simulink model "HPP"  (R2026a)
settings: Solver=ode1  StopTime=p.sim.Tstop  FixedStep=HPP_Tnet
model workspace (MAT data in the model file):
  HPP_Tnet = 0.001
  HPP_Ts = 0.001
  HPP_delays = 1
  HPP_f0 = 50
  HPP_network = 1
  HPP_simscape = 1
  buildInfo : object (value not decoded)
undefined symbols (not defined in the file): p
libraries: ee_lib x57, nesl_utility x29, fl_lib x6
(part 4 of 5)

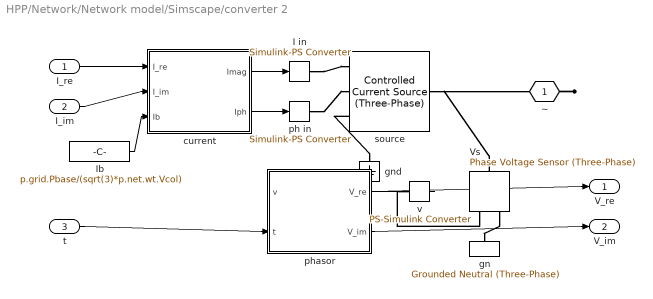
== system HPP/Network/Network model/Simscape/converter 2 ==
  I_re : Inport
  I_im : Inport  Port=2
  t : Inport  Port=3
  I in : nesl_utility/Simulink-PS Converter  PhysicalDomain=network_engine_domain  SubClassName=ps_input  LeftPortType=input  RightPortType=output  PseudoPeriodic=off  Frequencies=[]  NoiseDistribution=none  NoiseParameters=[]  Unit=A  AffineConversion=off  FilteringAndDerivatives=provide  SimscapeFilterOrder=1  InputFilterTimeConstant=0.001  UdotUserProvided=0
  Ib : Constant  Value=p.grid.Pbase/(sqrt(3)*p.net.wt.Vcol)
  Vs : ee_lib/Sensors & Transducers/Phase Voltage Sensor (Three-Phase)  port_option=ee.enum.threePhasePort.composite
  current : MATLAB Function  TreatAsAtomicUnit=on
  gn : ee_lib/Connectors & References/Grounded Neutral (Three-Phase)  port_option=ee.enum.threePhasePort.composite
  gnd : fl_lib/Electrical/Electrical Elements/Electrical Reference
  ph in : nesl_utility/Simulink-PS Converter  PhysicalDomain=network_engine_domain  SubClassName=ps_input  LeftPortType=input  RightPortType=output  PseudoPeriodic=off  Frequencies=[]  NoiseDistribution=none  NoiseParameters=[]  Unit=rad  AffineConversion=off  FilteringAndDerivatives=provide  SimscapeFilterOrder=1  InputFilterTimeConstant=0.001  UdotUserProvided=0
  phasor : Subsystem
  source : ee_lib/Sources/Controlled Current Source (Three-Phase)  port_option=ee.enum.threePhasePort.composite  input_option=ee.enum.inputType.singleFreqAC  FRated=HPP_f0 Hz  G_parasitic=0 1/Ohm
  v : nesl_utility/PS-Simulink Converter  PhysicalDomain=network_engine_domain  SubClassName=ps_output  LeftPortType=input  RightPortType=output  PseudoPeriodic=off  Frequencies=[]  VectorFormat=inherit  Unit=inherit  AffineConversion=off
  ~ : PMIOPort  Side=Right
  V_re : Outport
  V_im : Outport  Port=2
  wires:
  I_re/1 -> current/1(I_re)
  I_im/1 -> current/2(I_im)
  Ib/1 -> current/3(Ib)
  current/1(Imag) -> I in/1
  current/2(Iph) -> ph in/1
  v/1 -> phasor/1(v)
  t/1 -> phasor/2(t)
  phasor/1(V_re) -> V_re/1
  phasor/2(V_im) -> V_im/1
  connections:
  I in/RConn1 -- source/LConn1
  ph in/RConn1 -- source/LConn2
  source/LConn3 -- gnd/LConn1
  ~/RConn1 -- source/RConn1 -- Vs/LConn1
  Vs/RConn2 -- gn/LConn1
  Vs/RConn1 -- v/LConn1

== system HPP/Network/Network model/Simscape/converter 3 ==
  I_re : Inport
  I_im : Inport  Port=2
  t : Inport  Port=3
  I in : nesl_utility/Simulink-PS Converter  PhysicalDomain=network_engine_domain  SubClassName=ps_input  LeftPortType=input  RightPortType=output  PseudoPeriodic=off  Frequencies=[]  NoiseDistribution=none  NoiseParameters=[]  Unit=A  AffineConversion=off  FilteringAndDerivatives=provide  SimscapeFilterOrder=1  InputFilterTimeConstant=0.001  UdotUserProvided=0
  Ib : Constant  Value=p.grid.Pbase/(sqrt(3)*p.net.pv.Vcol)
  Vs : ee_lib/Sensors & Transducers/Phase Voltage Sensor (Three-Phase)  port_option=ee.enum.threePhasePort.composite
  current : MATLAB Function  TreatAsAtomicUnit=on
  gn : ee_lib/Connectors & References/Grounded Neutral (Three-Phase)  port_option=ee.enum.threePhasePort.composite
  gnd : fl_lib/Electrical/Electrical Elements/Electrical Reference
  ph in : nesl_utility/Simulink-PS Converter  PhysicalDomain=network_engine_domain  SubClassName=ps_input  LeftPortType=input  RightPortType=output  PseudoPeriodic=off  Frequencies=[]  NoiseDistribution=none  NoiseParameters=[]  Unit=rad  AffineConversion=off  FilteringAndDerivatives=provide  SimscapeFilterOrder=1  InputFilterTimeConstant=0.001  UdotUserProvided=0
  phasor : Subsystem
  source : ee_lib/Sources/Controlled Current Source (Three-Phase)  port_option=ee.enum.threePhasePort.composite  input_option=ee.enum.inputType.singleFreqAC  FRated=HPP_f0 Hz  G_parasitic=0 1/Ohm
  v : nesl_utility/PS-Simulink Converter  PhysicalDomain=network_engine_domain  SubClassName=ps_output  LeftPortType=input  RightPortType=output  PseudoPeriodic=off  Frequencies=[]  VectorFormat=inherit  Unit=inherit  AffineConversion=off
  ~ : PMIOPort  Side=Right
  V_re : Outport
  V_im : Outport  Port=2
  wires:
  I_re/1 -> current/1(I_re)
  I_im/1 -> current/2(I_im)
  Ib/1 -> current/3(Ib)
  current/1(Imag) -> I in/1
  current/2(Iph) -> ph in/1
  v/1 -> phasor/1(v)
  t/1 -> phasor/2(t)
  phasor/1(V_re) -> V_re/1
  phasor/2(V_im) -> V_im/1
  connections:
  I in/RConn1 -- source/LConn1
  ph in/RConn1 -- source/LConn2
  source/LConn3 -- gnd/LConn1
  ~/RConn1 -- source/RConn1 -- Vs/LConn1
  Vs/RConn2 -- gn/LConn1
  Vs/RConn1 -- v/LConn1

== system HPP/Network/Network model/Simscape/converter 4 ==
  I_re : Inport
  I_im : Inport  Port=2
  t : Inport  Port=3
  I in : nesl_utility/Simulink-PS Converter  PhysicalDomain=network_engine_domain  SubClassName=ps_input  LeftPortType=input  RightPortType=output  PseudoPeriodic=off  Frequencies=[]  NoiseDistribution=none  NoiseParameters=[]  Unit=A  AffineConversion=off  FilteringAndDerivatives=provide  SimscapeFilterOrder=1  InputFilterTimeConstant=0.001  UdotUserProvided=0
  Ib : Constant  Value=p.grid.Pbase/(sqrt(3)*p.net.pv.Vcol)
  Vs : ee_lib/Sensors & Transducers/Phase Voltage Sensor (Three-Phase)  port_option=ee.enum.threePhasePort.composite
  current : MATLAB Function  TreatAsAtomicUnit=on
  gn : ee_lib/Connectors & References/Grounded Neutral (Three-Phase)  port_option=ee.enum.threePhasePort.composite
  gnd : fl_lib/Electrical/Electrical Elements/Electrical Reference
  ph in : nesl_utility/Simulink-PS Converter  PhysicalDomain=network_engine_domain  SubClassName=ps_input  LeftPortType=input  RightPortType=output  PseudoPeriodic=off  Frequencies=[]  NoiseDistribution=none  NoiseParameters=[]  Unit=rad  AffineConversion=off  FilteringAndDerivatives=provide  SimscapeFilterOrder=1  InputFilterTimeConstant=0.001  UdotUserProvided=0
  phasor : Subsystem
  source : ee_lib/Sources/Controlled Current Source (Three-Phase)  port_option=ee.enum.threePhasePort.composite  input_option=ee.enum.inputType.singleFreqAC  FRated=HPP_f0 Hz  G_parasitic=0 1/Ohm
  v : nesl_utility/PS-Simulink Converter  PhysicalDomain=network_engine_domain  SubClassName=ps_output  LeftPortType=input  RightPortType=output  PseudoPeriodic=off  Frequencies=[]  VectorFormat=inherit  Unit=inherit  AffineConversion=off
  ~ : PMIOPort  Side=Right
  V_re : Outport
  V_im : Outport  Port=2
  wires:
  I_re/1 -> current/1(I_re)
  I_im/1 -> current/2(I_im)
  Ib/1 -> current/3(Ib)
  current/1(Imag) -> I in/1
  current/2(Iph) -> ph in/1
  v/1 -> phasor/1(v)
  t/1 -> phasor/2(t)
  phasor/1(V_re) -> V_re/1
  phasor/2(V_im) -> V_im/1
  connections:
  I in/RConn1 -- source/LConn1
  ph in/RConn1 -- source/LConn2
  source/LConn3 -- gnd/LConn1
  ~/RConn1 -- source/RConn1 -- Vs/LConn1
  Vs/RConn2 -- gn/LConn1
  Vs/RConn1 -- v/LConn1

== system HPP/Network/Network model/Simscape/converter 5 ==
  I_re : Inport
  I_im : Inport  Port=2
  t : Inport  Port=3
  I in : nesl_utility/Simulink-PS Converter  PhysicalDomain=network_engine_domain  SubClassName=ps_input  LeftPortType=input  RightPortType=output  PseudoPeriodic=off  Frequencies=[]  NoiseDistribution=none  NoiseParameters=[]  Unit=A  AffineConversion=off  FilteringAndDerivatives=provide  SimscapeFilterOrder=1  InputFilterTimeConstant=0.001  UdotUserProvided=0
  Ib : Constant  Value=p.grid.Pbase/(sqrt(3)*p.net.bess.Vcol)
  Vs : ee_lib/Sensors & Transducers/Phase Voltage Sensor (Three-Phase)  port_option=ee.enum.threePhasePort.composite
  current : MATLAB Function  TreatAsAtomicUnit=on
  gn : ee_lib/Connectors & References/Grounded Neutral (Three-Phase)  port_option=ee.enum.threePhasePort.composite
  gnd : fl_lib/Electrical/Electrical Elements/Electrical Reference
  ph in : nesl_utility/Simulink-PS Converter  PhysicalDomain=network_engine_domain  SubClassName=ps_input  LeftPortType=input  RightPortType=output  PseudoPeriodic=off  Frequencies=[]  NoiseDistribution=none  NoiseParameters=[]  Unit=rad  AffineConversion=off  FilteringAndDerivatives=provide  SimscapeFilterOrder=1  InputFilterTimeConstant=0.001  UdotUserProvided=0
  phasor : Subsystem
  source : ee_lib/Sources/Controlled Current Source (Three-Phase)  port_option=ee.enum.threePhasePort.composite  input_option=ee.enum.inputType.singleFreqAC  FRated=HPP_f0 Hz  G_parasitic=0 1/Ohm
  v : nesl_utility/PS-Simulink Converter  PhysicalDomain=network_engine_domain  SubClassName=ps_output  LeftPortType=input  RightPortType=output  PseudoPeriodic=off  Frequencies=[]  VectorFormat=inherit  Unit=inherit  AffineConversion=off
  ~ : PMIOPort  Side=Right
  V_re : Outport
  V_im : Outport  Port=2
  wires:
  I_re/1 -> current/1(I_re)
  I_im/1 -> current/2(I_im)
  Ib/1 -> current/3(Ib)
  current/1(Imag) -> I in/1
  current/2(Iph) -> ph in/1
  v/1 -> phasor/1(v)
  t/1 -> phasor/2(t)
  phasor/1(V_re) -> V_re/1
  phasor/2(V_im) -> V_im/1
  connections:
  I in/RConn1 -- source/LConn1
  ph in/RConn1 -- source/LConn2
  source/LConn3 -- gnd/LConn1
  ~/RConn1 -- source/RConn1 -- Vs/LConn1
  Vs/RConn2 -- gn/LConn1
  Vs/RConn1 -- v/LConn1

== system HPP/Network/Network model/Simscape/feeder 1 ==
  Ca : ee_lib/Passive/RLC Assemblies/RLC (Three-Phase)  port_option=ee.enum.threePhasePort.composite  component_structure=ee.enum.rlc.structure.C  R=1 Ohm  L=1e-3 H  C=p.net.wt.cable.C*p.net.wt.cable.len1*p.net.wt.cable.nPar/2 F  R_parasitic=0 Ohm  G_parasitic=0 1/Ohm  IL_specify=off  IL_priority=High  IL=[0, 0, 0] A  IL_nominal_specify=off  IL_nominal_value=1  IL_nominal_unit=A  VC_specify=off  VC_priority=High  VC=[0, 0, 0] V  VC_nominal_specify=off  VC_nominal_value=1  VC_nominal_unit=V
  Cb : ee_lib/Passive/RLC Assemblies/RLC (Three-Phase)  port_option=ee.enum.threePhasePort.composite  component_structure=ee.enum.rlc.structure.C  R=1 Ohm  L=1e-3 H  C=p.net.wt.cable.C*p.net.wt.cable.len1*p.net.wt.cable.nPar/2 F  R_parasitic=0 Ohm  G_parasitic=0 1/Ohm  IL_specify=off  IL_priority=High  IL=[0, 0, 0] A  IL_nominal_specify=off  IL_nominal_value=1  IL_nominal_unit=A  VC_specify=off  VC_priority=High  VC=[0, 0, 0] V  VC_nominal_specify=off  VC_nominal_value=1  VC_nominal_unit=V
  gnd a : ee_lib/Connectors & References/Grounded Neutral (Three-Phase)  port_option=ee.enum.threePhasePort.composite
  gnd b : ee_lib/Connectors & References/Grounded Neutral (Three-Phase)  port_option=ee.enum.threePhasePort.composite
  series : ee_lib/Passive/RLC Assemblies/RLC (Three-Phase)  port_option=ee.enum.threePhasePort.composite  component_structure=ee.enum.rlc.structure.SeriesRL  R=p.net.wt.cable.R*p.net.wt.cable.len1/p.net.wt.cable.nPar Ohm  L=p.net.wt.cable.X*p.net.wt.cable.len1/(2*pi*p.grid.f0)/p.net.wt.cable.nPar H  C=1e-6 F  R_parasitic=0 Ohm  G_parasitic=0 1/Ohm  IL_specify=off  IL_priority=High  IL=[0, 0, 0] A  IL_nominal_specify=off  IL_nominal_value=1  IL_nominal_unit=A  VC_specify=off  VC_priority=High  VC=[0, 0, 0] V  VC_nominal_specify=off  VC_nominal_value=1  VC_nominal_unit=V
  a : PMIOPort  Side=Left
  b : PMIOPort  Port=2  Side=Right
  connections:
  series/LConn1 -- a/RConn1 -- Ca/LConn1
  series/RConn1 -- b/RConn1 -- Cb/LConn1
  Ca/RConn1 -- gnd a/LConn1
  Cb/RConn1 -- gnd b/LConn1

== system HPP/Network/Network model/Simscape/feeder 2 ==
  Ca : ee_lib/Passive/RLC Assemblies/RLC (Three-Phase)  port_option=ee.enum.threePhasePort.composite  component_structure=ee.enum.rlc.structure.C  R=1 Ohm  L=1e-3 H  C=p.net.wt.cable.C*p.net.wt.cable.len*p.net.wt.cable.nPar/2 F  R_parasitic=0 Ohm  G_parasitic=0 1/Ohm  IL_specify=off  IL_priority=High  IL=[0, 0, 0] A  IL_nominal_specify=off  IL_nominal_value=1  IL_nominal_unit=A  VC_specify=off  VC_priority=High  VC=[0, 0, 0] V  VC_nominal_specify=off  VC_nominal_value=1  VC_nominal_unit=V
  Cb : ee_lib/Passive/RLC Assemblies/RLC (Three-Phase)  port_option=ee.enum.threePhasePort.composite  component_structure=ee.enum.rlc.structure.C  R=1 Ohm  L=1e-3 H  C=p.net.wt.cable.C*p.net.wt.cable.len*p.net.wt.cable.nPar/2 F  R_parasitic=0 Ohm  G_parasitic=0 1/Ohm  IL_specify=off  IL_priority=High  IL=[0, 0, 0] A  IL_nominal_specify=off  IL_nominal_value=1  IL_nominal_unit=A  VC_specify=off  VC_priority=High  VC=[0, 0, 0] V  VC_nominal_specify=off  VC_nominal_value=1  VC_nominal_unit=V
  gnd a : ee_lib/Connectors & References/Grounded Neutral (Three-Phase)  port_option=ee.enum.threePhasePort.composite
  gnd b : ee_lib/Connectors & References/Grounded Neutral (Three-Phase)  port_option=ee.enum.threePhasePort.composite
  series : ee_lib/Passive/RLC Assemblies/RLC (Three-Phase)  port_option=ee.enum.threePhasePort.composite  component_structure=ee.enum.rlc.structure.SeriesRL  R=p.net.wt.cable.R*p.net.wt.cable.len/p.net.wt.cable.nPar Ohm  L=p.net.wt.cable.X*p.net.wt.cable.len/(2*pi*p.grid.f0)/p.net.wt.cable.nPar H  C=1e-6 F  R_parasitic=0 Ohm  G_parasitic=0 1/Ohm  IL_specify=off  IL_priority=High  IL=[0, 0, 0] A  IL_nominal_specify=off  IL_nominal_value=1  IL_nominal_unit=A  VC_specify=off  VC_priority=High  VC=[0, 0, 0] V  VC_nominal_specify=off  VC_nominal_value=1  VC_nominal_unit=V
  a : PMIOPort  Side=Left
  b : PMIOPort  Port=2  Side=Right
  connections:
  series/LConn1 -- a/RConn1 -- Ca/LConn1
  series/RConn1 -- b/RConn1 -- Cb/LConn1
  Ca/RConn1 -- gnd a/LConn1
  Cb/RConn1 -- gnd b/LConn1

== system HPP/Network/Network model/Simscape/feeder 3 ==
  Ca : ee_lib/Passive/RLC Assemblies/RLC (Three-Phase)  port_option=ee.enum.threePhasePort.composite  component_structure=ee.enum.rlc.structure.C  R=1 Ohm  L=1e-3 H  C=p.net.pv.cable.C*p.net.pv.cable.len1*p.net.pv.cable.nPar/2 F  R_parasitic=0 Ohm  G_parasitic=0 1/Ohm  IL_specify=off  IL_priority=High  IL=[0, 0, 0] A  IL_nominal_specify=off  IL_nominal_value=1  IL_nominal_unit=A  VC_specify=off  VC_priority=High  VC=[0, 0, 0] V  VC_nominal_specify=off  VC_nominal_value=1  VC_nominal_unit=V
  Cb : ee_lib/Passive/RLC Assemblies/RLC (Three-Phase)  port_option=ee.enum.threePhasePort.composite  component_structure=ee.enum.rlc.structure.C  R=1 Ohm  L=1e-3 H  C=p.net.pv.cable.C*p.net.pv.cable.len1*p.net.pv.cable.nPar/2 F  R_parasitic=0 Ohm  G_parasitic=0 1/Ohm  IL_specify=off  IL_priority=High  IL=[0, 0, 0] A  IL_nominal_specify=off  IL_nominal_value=1  IL_nominal_unit=A  VC_specify=off  VC_priority=High  VC=[0, 0, 0] V  VC_nominal_specify=off  VC_nominal_value=1  VC_nominal_unit=V
  gnd a : ee_lib/Connectors & References/Grounded Neutral (Three-Phase)  port_option=ee.enum.threePhasePort.composite
  gnd b : ee_lib/Connectors & References/Grounded Neutral (Three-Phase)  port_option=ee.enum.threePhasePort.composite
  series : ee_lib/Passive/RLC Assemblies/RLC (Three-Phase)  port_option=ee.enum.threePhasePort.composite  component_structure=ee.enum.rlc.structure.SeriesRL  R=p.net.pv.cable.R*p.net.pv.cable.len1/p.net.pv.cable.nPar Ohm  L=p.net.pv.cable.X*p.net.pv.cable.len1/(2*pi*p.grid.f0)/p.net.pv.cable.nPar H  C=1e-6 F  R_parasitic=0 Ohm  G_parasitic=0 1/Ohm  IL_specify=off  IL_priority=High  IL=[0, 0, 0] A  IL_nominal_specify=off  IL_nominal_value=1  IL_nominal_unit=A  VC_specify=off  VC_priority=High  VC=[0, 0, 0] V  VC_nominal_specify=off  VC_nominal_value=1  VC_nominal_unit=V
  a : PMIOPort  Side=Left
  b : PMIOPort  Port=2  Side=Right
  connections:
  series/LConn1 -- a/RConn1 -- Ca/LConn1
  series/RConn1 -- b/RConn1 -- Cb/LConn1
  Ca/RConn1 -- gnd a/LConn1
  Cb/RConn1 -- gnd b/LConn1

== system HPP/Network/Network model/Simscape/feeder 4 ==
  Ca : ee_lib/Passive/RLC Assemblies/RLC (Three-Phase)  port_option=ee.enum.threePhasePort.composite  component_structure=ee.enum.rlc.structure.C  R=1 Ohm  L=1e-3 H  C=p.net.pv.cable.C*p.net.pv.cable.len1*p.net.pv.cable.nPar/2 F  R_parasitic=0 Ohm  G_parasitic=0 1/Ohm  IL_specify=off  IL_priority=High  IL=[0, 0, 0] A  IL_nominal_specify=off  IL_nominal_value=1  IL_nominal_unit=A  VC_specify=off  VC_priority=High  VC=[0, 0, 0] V  VC_nominal_specify=off  VC_nominal_value=1  VC_nominal_unit=V
  Cb : ee_lib/Passive/RLC Assemblies/RLC (Three-Phase)  port_option=ee.enum.threePhasePort.composite  component_structure=ee.enum.rlc.structure.C  R=1 Ohm  L=1e-3 H  C=p.net.pv.cable.C*p.net.pv.cable.len1*p.net.pv.cable.nPar/2 F  R_parasitic=0 Ohm  G_parasitic=0 1/Ohm  IL_specify=off  IL_priority=High  IL=[0, 0, 0] A  IL_nominal_specify=off  IL_nominal_value=1  IL_nominal_unit=A  VC_specify=off  VC_priority=High  VC=[0, 0, 0] V  VC_nominal_specify=off  VC_nominal_value=1  VC_nominal_unit=V
  gnd a : ee_lib/Connectors & References/Grounded Neutral (Three-Phase)  port_option=ee.enum.threePhasePort.composite
  gnd b : ee_lib/Connectors & References/Grounded Neutral (Three-Phase)  port_option=ee.enum.threePhasePort.composite
  series : ee_lib/Passive/RLC Assemblies/RLC (Three-Phase)  port_option=ee.enum.threePhasePort.composite  component_structure=ee.enum.rlc.structure.SeriesRL  R=p.net.pv.cable.R*p.net.pv.cable.len1/p.net.pv.cable.nPar Ohm  L=p.net.pv.cable.X*p.net.pv.cable.len1/(2*pi*p.grid.f0)/p.net.pv.cable.nPar H  C=1e-6 F  R_parasitic=0 Ohm  G_parasitic=0 1/Ohm  IL_specify=off  IL_priority=High  IL=[0, 0, 0] A  IL_nominal_specify=off  IL_nominal_value=1  IL_nominal_unit=A  VC_specify=off  VC_priority=High  VC=[0, 0, 0] V  VC_nominal_specify=off  VC_nominal_value=1  VC_nominal_unit=V
  a : PMIOPort  Side=Left
  b : PMIOPort  Port=2  Side=Right
  connections:
  series/LConn1 -- a/RConn1 -- Ca/LConn1
  series/RConn1 -- b/RConn1 -- Cb/LConn1
  Ca/RConn1 -- gnd a/LConn1
  Cb/RConn1 -- gnd b/LConn1

== system HPP/Network/Network model/Simscape/feeder 5 ==
  Ca : ee_lib/Passive/RLC Assemblies/RLC (Three-Phase)  port_option=ee.enum.threePhasePort.composite  component_structure=ee.enum.rlc.structure.C  R=1 Ohm  L=1e-3 H  C=p.net.bess.cable.C*p.net.bess.cable.len1*p.net.bess.cable.nPar/2 F  R_parasitic=0 Ohm  G_parasitic=0 1/Ohm  IL_specify=off  IL_priority=High  IL=[0, 0, 0] A  IL_nominal_specify=off  IL_nominal_value=1  IL_nominal_unit=A  VC_specify=off  VC_priority=High  VC=[0, 0, 0] V  VC_nominal_specify=off  VC_nominal_value=1  VC_nominal_unit=V
  Cb : ee_lib/Passive/RLC Assemblies/RLC (Three-Phase)  port_option=ee.enum.threePhasePort.composite  component_structure=ee.enum.rlc.structure.C  R=1 Ohm  L=1e-3 H  C=p.net.bess.cable.C*p.net.bess.cable.len1*p.net.bess.cable.nPar/2 F  R_parasitic=0 Ohm  G_parasitic=0 1/Ohm  IL_specify=off  IL_priority=High  IL=[0, 0, 0] A  IL_nominal_specify=off  IL_nominal_value=1  IL_nominal_unit=A  VC_specify=off  VC_priority=High  VC=[0, 0, 0] V  VC_nominal_specify=off  VC_nominal_value=1  VC_nominal_unit=V
  gnd a : ee_lib/Connectors & References/Grounded Neutral (Three-Phase)  port_option=ee.enum.threePhasePort.composite
  gnd b : ee_lib/Connectors & References/Grounded Neutral (Three-Phase)  port_option=ee.enum.threePhasePort.composite
  series : ee_lib/Passive/RLC Assemblies/RLC (Three-Phase)  port_option=ee.enum.threePhasePort.composite  component_structure=ee.enum.rlc.structure.SeriesRL  R=p.net.bess.cable.R*p.net.bess.cable.len1/p.net.bess.cable.nPar Ohm  L=p.net.bess.cable.X*p.net.bess.cable.len1/(2*pi*p.grid.f0)/p.net.bess.cable.nPar H  C=1e-6 F  R_parasitic=0 Ohm  G_parasitic=0 1/Ohm  IL_specify=off  IL_priority=High  IL=[0, 0, 0] A  IL_nominal_specify=off  IL_nominal_value=1  IL_nominal_unit=A  VC_specify=off  VC_priority=High  VC=[0, 0, 0] V  VC_nominal_specify=off  VC_nominal_value=1  VC_nominal_unit=V
  a : PMIOPort  Side=Left
  b : PMIOPort  Port=2  Side=Right
  connections:
  series/LConn1 -- a/RConn1 -- Ca/LConn1
  series/RConn1 -- b/RConn1 -- Cb/LConn1
  Ca/RConn1 -- gnd a/LConn1
  Cb/RConn1 -- gnd b/LConn1

== system HPP/Network/Network model/Simscape/solver ==
  note: 1) Add Subsystem or Model blocks as valid variant choices.
      | 2) You cannot connect blocks at this level. At simulation, connectivity is automatically
      | determined, based on the active variant and port name matching.
  EMT : Subsystem  VariantControl=HPP_simscape == 2
  Phasor : Subsystem  VariantControl=HPP_simscape == 1
  ~ : PMIOPort  Side=Right

== system HPP/Network/Network model/Simscape/spp meter ==
  P hold : ZeroOrderHold  SampleTime=HPP_Ts
  P out : nesl_utility/PS-Simulink Converter  PhysicalDomain=network_engine_domain  SubClassName=ps_output  LeftPortType=input  RightPortType=output  PseudoPeriodic=off  Frequencies=[]  VectorFormat=inherit  Unit=inherit  AffineConversion=off
  PQ : ee_lib/Sensors & Transducers/Power Sensor (Three-Phase)  port_option=ee.enum.threePhasePort.composite  load_type=ee.enum.passive.type_balanced.balanced  f0=HPP_f0 Hz
  Q hold : ZeroOrderHold  SampleTime=HPP_Ts
  Q out : nesl_utility/PS-Simulink Converter  PhysicalDomain=network_engine_domain  SubClassName=ps_output  LeftPortType=input  RightPortType=output  PseudoPeriodic=off  Frequencies=[]  VectorFormat=inherit  Unit=inherit  AffineConversion=off
  a : PMIOPort  Side=Left
  b : PMIOPort  Port=2  Side=Right
  P : Outport
  Q : Outport  Port=2
  wires:
  P out/1 -> P hold/1
  P hold/1 -> P/1
  Q out/1 -> Q hold/1
  Q hold/1 -> Q/1
  connections:
  a/RConn1 -- PQ/LConn1
  b/RConn1 -- PQ/RConn1
  PQ/LConn2 -- P out/LConn1
  PQ/LConn3 -- Q out/LConn1

== system HPP/Network/Network model/Simscape/wpp meter ==
  P hold : ZeroOrderHold  SampleTime=HPP_Ts
  P out : nesl_utility/PS-Simulink Converter  PhysicalDomain=network_engine_domain  SubClassName=ps_output  LeftPortType=input  RightPortType=output  PseudoPeriodic=off  Frequencies=[]  VectorFormat=inherit  Unit=inherit  AffineConversion=off
  PQ : ee_lib/Sensors & Transducers/Power Sensor (Three-Phase)  port_option=ee.enum.threePhasePort.composite  load_type=ee.enum.passive.type_balanced.balanced  f0=HPP_f0 Hz
  Q hold : ZeroOrderHold  SampleTime=HPP_Ts
  Q out : nesl_utility/PS-Simulink Converter  PhysicalDomain=network_engine_domain  SubClassName=ps_output  LeftPortType=input  RightPortType=output  PseudoPeriodic=off  Frequencies=[]  VectorFormat=inherit  Unit=inherit  AffineConversion=off
  a : PMIOPort  Side=Left
  b : PMIOPort  Port=2  Side=Right
  P : Outport
  Q : Outport  Port=2
  wires:
  P out/1 -> P hold/1
  P hold/1 -> P/1
  Q out/1 -> Q hold/1
  Q hold/1 -> Q/1
  connections:
  a/RConn1 -- PQ/LConn1
  b/RConn1 -- PQ/RConn1
  PQ/LConn2 -- P out/LConn1
  PQ/LConn3 -- Q out/LConn1

== system HPP/PV plant/P_avail_k link/delay 3/Fixed ==
  u : Inport
  Delay : Delay  DelayLength=p.comm.steps.meas_plant  InitialCondition=0  SampleTime=p.sim.Ts
  y : Outport
  wires:
  Delay/1 -> y/1
  u/1 -> Delay/1

== system HPP/PV plant/P_avail_k link/delay 3/Variable ==
  u : Inport
  Delay : Delay  DelayLengthSource=Input port  DelayLengthUpperLimit=round(p.comm.maxDelay/p.sim.Ts)  InitialCondition=0  SampleTime=p.sim.Ts
      settings: InputPortMap=u0,p1
  steps : Constant  Value=p.comm.steps.meas_plant  OutDataTypeStr=double  SampleTime=p.sim.Ts
  y : Outport
  wires:
  Delay/1 -> y/1
  u/1 -> Delay/1
  steps/1 -> Delay/2

== system HPP/PV plant/P_meas link/delay 3/Fixed ==
  u : Inport
  Delay : Delay  DelayLength=p.comm.steps.meas_plant  InitialCondition=0  SampleTime=p.sim.Ts
  y : Outport
  wires:
  Delay/1 -> y/1
  u/1 -> Delay/1

== system HPP/PV plant/P_meas link/delay 3/Variable ==
  u : Inport
  Delay : Delay  DelayLengthSource=Input port  DelayLengthUpperLimit=round(p.comm.maxDelay/p.sim.Ts)  InitialCondition=0  SampleTime=p.sim.Ts
      settings: InputPortMap=u0,p1
  steps : Constant  Value=p.comm.steps.meas_plant  OutDataTypeStr=double  SampleTime=p.sim.Ts
  y : Outport
  wires:
  u/1 -> Delay/1
  steps/1 -> Delay/2
  Delay/1 -> y/1

== system HPP/PV plant/P_set link/delay 1/Fixed ==
  u : Inport
  Delay : Delay  DelayLength=p.comm.steps.hppc_to_plant  InitialCondition=0  SampleTime=p.sim.Ts
  y : Outport
  wires:
  u/1 -> Delay/1
  Delay/1 -> y/1

== system HPP/PV plant/P_set link/delay 1/Variable ==
  u : Inport
  Delay : Delay  DelayLengthSource=Input port  DelayLengthUpperLimit=round(p.comm.maxDelay/p.sim.Ts)  InitialCondition=0  SampleTime=p.sim.Ts
      settings: InputPortMap=u0,p1
  steps : Constant  Value=p.comm.steps.hppc_to_plant  OutDataTypeStr=double  SampleTime=p.sim.Ts
  y : Outport
  wires:
  u/1 -> Delay/1
  steps/1 -> Delay/2
  Delay/1 -> y/1

== system HPP/PV plant/P_set_k link/delay 1/Fixed ==
  u : Inport
  Delay : Delay  DelayLength=p.comm.steps.plant_to_asset  InitialCondition=0  SampleTime=p.sim.Ts
  y : Outport
  wires:
  Delay/1 -> y/1
  u/1 -> Delay/1

== system HPP/PV plant/P_set_k link/delay 1/Variable ==
  u : Inport
  Delay : Delay  DelayLengthSource=Input port  DelayLengthUpperLimit=round(p.comm.maxDelay/p.sim.Ts)  InitialCondition=0  SampleTime=p.sim.Ts
      settings: InputPortMap=u0,p1
  steps : Constant  Value=p.comm.steps.plant_to_asset  OutDataTypeStr=double  SampleTime=p.sim.Ts
  y : Outport
  wires:
  u/1 -> Delay/1
  steps/1 -> Delay/2
  Delay/1 -> y/1

== system HPP/PV plant/Q_meas link/delay 3/Fixed ==
  u : Inport
  Delay : Delay  DelayLength=p.comm.steps.meas_plant  InitialCondition=0  SampleTime=p.sim.Ts
  y : Outport
  wires:
  u/1 -> Delay/1
  Delay/1 -> y/1

== system HPP/PV plant/Q_meas link/delay 3/Variable ==
  u : Inport
  Delay : Delay  DelayLengthSource=Input port  DelayLengthUpperLimit=round(p.comm.maxDelay/p.sim.Ts)  InitialCondition=0  SampleTime=p.sim.Ts
      settings: InputPortMap=u0,p1
  steps : Constant  Value=p.comm.steps.meas_plant  OutDataTypeStr=double  SampleTime=p.sim.Ts
  y : Outport
  wires:
  u/1 -> Delay/1
  steps/1 -> Delay/2
  Delay/1 -> y/1

== system HPP/PV plant/Q_set link/delay 1/Fixed ==
  u : Inport
  Delay : Delay  DelayLength=p.comm.steps.hppc_to_plant  InitialCondition=0  SampleTime=p.sim.Ts
  y : Outport
  wires:
  u/1 -> Delay/1
  Delay/1 -> y/1

== system HPP/PV plant/Q_set link/delay 1/Variable ==
  u : Inport
  Delay : Delay  DelayLengthSource=Input port  DelayLengthUpperLimit=round(p.comm.maxDelay/p.sim.Ts)  InitialCondition=0  SampleTime=p.sim.Ts
      settings: InputPortMap=u0,p1
  steps : Constant  Value=p.comm.steps.hppc_to_plant  OutDataTypeStr=double  SampleTime=p.sim.Ts
  y : Outport
  wires:
  Delay/1 -> y/1
  u/1 -> Delay/1
  steps/1 -> Delay/2

== system HPP/PV plant/Q_set_k link/delay 1/Fixed ==
  u : Inport
  Delay : Delay  DelayLength=p.comm.steps.plant_to_asset  InitialCondition=0  SampleTime=p.sim.Ts
  y : Outport
  wires:
  u/1 -> Delay/1
  Delay/1 -> y/1

== system HPP/PV plant/Q_set_k link/delay 1/Variable ==
  u : Inport
  Delay : Delay  DelayLengthSource=Input port  DelayLengthUpperLimit=round(p.comm.maxDelay/p.sim.Ts)  InitialCondition=0  SampleTime=p.sim.Ts
      settings: InputPortMap=u0,p1
  steps : Constant  Value=p.comm.steps.plant_to_asset  OutDataTypeStr=double  SampleTime=p.sim.Ts
  y : Outport
  wires:
  u/1 -> Delay/1
  steps/1 -> Delay/2
  Delay/1 -> y/1

== system HPP/PV plant/V_meas link/delay 2/Fixed ==
  u : Inport
  Delay : Delay  DelayLength=p.comm.steps.meas_plant  InitialCondition=1  SampleTime=p.sim.Ts
  y : Outport
  wires:
  u/1 -> Delay/1
  Delay/1 -> y/1

== system HPP/PV plant/V_meas link/delay 2/Variable ==
  u : Inport
  Delay : Delay  DelayLengthSource=Input port  DelayLengthUpperLimit=round(p.comm.maxDelay/p.sim.Ts)  InitialCondition=1  SampleTime=p.sim.Ts
      settings: InputPortMap=u0,p1
  steps : Constant  Value=p.comm.steps.meas_plant  OutDataTypeStr=double  SampleTime=p.sim.Ts
  y : Outport
  wires:
  Delay/1 -> y/1
  u/1 -> Delay/1
  steps/1 -> Delay/2

== system HPP/Wind plant/P_avail_k link/delay 3/Fixed ==
  u : Inport
  Delay : Delay  DelayLength=p.comm.steps.meas_plant  InitialCondition=0  SampleTime=p.sim.Ts
  y : Outport
  wires:
  u/1 -> Delay/1
  Delay/1 -> y/1

== system HPP/Wind plant/P_avail_k link/delay 3/Variable ==
  u : Inport
  Delay : Delay  DelayLengthSource=Input port  DelayLengthUpperLimit=round(p.comm.maxDelay/p.sim.Ts)  InitialCondition=0  SampleTime=p.sim.Ts
      settings: InputPortMap=u0,p1
  steps : Constant  Value=p.comm.steps.meas_plant  OutDataTypeStr=double  SampleTime=p.sim.Ts
  y : Outport
  wires:
  u/1 -> Delay/1
  steps/1 -> Delay/2
  Delay/1 -> y/1

== system HPP/Wind plant/P_meas link/delay 3/Fixed ==
  u : Inport
  Delay : Delay  DelayLength=p.comm.steps.meas_plant  InitialCondition=0  SampleTime=p.sim.Ts
  y : Outport
  wires:
  u/1 -> Delay/1
  Delay/1 -> y/1

== system HPP/Wind plant/P_meas link/delay 3/Variable ==
  u : Inport
  Delay : Delay  DelayLengthSource=Input port  DelayLengthUpperLimit=round(p.comm.maxDelay/p.sim.Ts)  InitialCondition=0  SampleTime=p.sim.Ts
      settings: InputPortMap=u0,p1
  steps : Constant  Value=p.comm.steps.meas_plant  OutDataTypeStr=double  SampleTime=p.sim.Ts
  y : Outport
  wires:
  Delay/1 -> y/1
  u/1 -> Delay/1
  steps/1 -> Delay/2

== system HPP/Wind plant/P_set link/delay 1/Fixed ==
  u : Inport
  Delay : Delay  DelayLength=p.comm.steps.hppc_to_plant  InitialCondition=0  SampleTime=p.sim.Ts
  y : Outport
  wires:
  u/1 -> Delay/1
  Delay/1 -> y/1

== system HPP/Wind plant/P_set link/delay 1/Variable ==
  u : Inport
  Delay : Delay  DelayLengthSource=Input port  DelayLengthUpperLimit=round(p.comm.maxDelay/p.sim.Ts)  InitialCondition=0  SampleTime=p.sim.Ts
      settings: InputPortMap=u0,p1
  steps : Constant  Value=p.comm.steps.hppc_to_plant  OutDataTypeStr=double  SampleTime=p.sim.Ts
  y : Outport
  wires:
  u/1 -> Delay/1
  steps/1 -> Delay/2
  Delay/1 -> y/1

== system HPP/Wind plant/P_set_k link/delay 1/Fixed ==
  u : Inport
  Delay : Delay  DelayLength=p.comm.steps.plant_to_asset  InitialCondition=0  SampleTime=p.sim.Ts
  y : Outport
  wires:
  u/1 -> Delay/1
  Delay/1 -> y/1

== system HPP/Wind plant/P_set_k link/delay 1/Variable ==
  u : Inport
  Delay : Delay  DelayLengthSource=Input port  DelayLengthUpperLimit=round(p.comm.maxDelay/p.sim.Ts)  InitialCondition=0  SampleTime=p.sim.Ts
      settings: InputPortMap=u0,p1
  steps : Constant  Value=p.comm.steps.plant_to_asset  OutDataTypeStr=double  SampleTime=p.sim.Ts
  y : Outport
  wires:
  Delay/1 -> y/1
  u/1 -> Delay/1
  steps/1 -> Delay/2

== system HPP/Wind plant/Q_meas link/delay 3/Fixed ==
  u : Inport
  Delay : Delay  DelayLength=p.comm.steps.meas_plant  InitialCondition=0  SampleTime=p.sim.Ts
  y : Outport
  wires:
  u/1 -> Delay/1
  Delay/1 -> y/1

== system HPP/Wind plant/Q_meas link/delay 3/Variable ==
  u : Inport
  Delay : Delay  DelayLengthSource=Input port  DelayLengthUpperLimit=round(p.comm.maxDelay/p.sim.Ts)  InitialCondition=0  SampleTime=p.sim.Ts
      settings: InputPortMap=u0,p1
  steps : Constant  Value=p.comm.steps.meas_plant  OutDataTypeStr=double  SampleTime=p.sim.Ts
  y : Outport
  wires:
  steps/1 -> Delay/2
  u/1 -> Delay/1
  Delay/1 -> y/1

== system HPP/Wind plant/Q_set link/delay 1/Fixed ==
  u : Inport
  Delay : Delay  DelayLength=p.comm.steps.hppc_to_plant  InitialCondition=0  SampleTime=p.sim.Ts
  y : Outport
  wires:
  u/1 -> Delay/1
  Delay/1 -> y/1

== system HPP/Wind plant/Q_set link/delay 1/Variable ==
  u : Inport
  Delay : Delay  DelayLengthSource=Input port  DelayLengthUpperLimit=round(p.comm.maxDelay/p.sim.Ts)  InitialCondition=0  SampleTime=p.sim.Ts
      settings: InputPortMap=u0,p1
  steps : Constant  Value=p.comm.steps.hppc_to_plant  OutDataTypeStr=double  SampleTime=p.sim.Ts
  y : Outport
  wires:
  Delay/1 -> y/1
  u/1 -> Delay/1
  steps/1 -> Delay/2

== system HPP/Wind plant/Q_set_k link/delay 1/Fixed ==
  u : Inport
  Delay : Delay  DelayLength=p.comm.steps.plant_to_asset  InitialCondition=0  SampleTime=p.sim.Ts
  y : Outport
  wires:
  Delay/1 -> y/1
  u/1 -> Delay/1

== system HPP/Wind plant/Q_set_k link/delay 1/Variable ==
  u : Inport
  Delay : Delay  DelayLengthSource=Input port  DelayLengthUpperLimit=round(p.comm.maxDelay/p.sim.Ts)  InitialCondition=0  SampleTime=p.sim.Ts
      settings: InputPortMap=u0,p1
  steps : Constant  Value=p.comm.steps.plant_to_asset  OutDataTypeStr=double  SampleTime=p.sim.Ts
  y : Outport
  wires:
  u/1 -> Delay/1
  steps/1 -> Delay/2
  Delay/1 -> y/1

== system HPP/Wind plant/V_meas link/delay 2/Fixed ==
  u : Inport
  Delay : Delay  DelayLength=p.comm.steps.meas_plant  InitialCondition=1  SampleTime=p.sim.Ts
  y : Outport
  wires:
  u/1 -> Delay/1
  Delay/1 -> y/1

== system HPP/Wind plant/V_meas link/delay 2/Variable ==
  u : Inport
  Delay : Delay  DelayLengthSource=Input port  DelayLengthUpperLimit=round(p.comm.maxDelay/p.sim.Ts)  InitialCondition=1  SampleTime=p.sim.Ts
      settings: InputPortMap=u0,p1
  steps : Constant  Value=p.comm.steps.meas_plant  OutDataTypeStr=double  SampleTime=p.sim.Ts
  y : Outport
  wires:
  u/1 -> Delay/1
  steps/1 -> Delay/2
  Delay/1 -> y/1

== system HPP/Network/Network model/Simscape/HPP bus voltage/phasor ==
  v : Inport
  t : Inport  Port=2
  Vn : Constant  Value=p.net.Vhpp
  filter : Subsystem  Description=Voltage phasor filter, chosen per run by HPP_simscape: None (1, phasor mode) or MAF (2, EMT: moving average over one cycle at p.sim.Ts, starting from the nominal phasor 1 + 0j pu).  Variant=on
  hold : ZeroOrderHold  SampleTime=HPP_Ts
  space phasor : MATLAB Function  TreatAsAtomicUnit=on
  w0 : Constant  Value=2*pi*p.grid.f0
  V_re : Outport
  V_im : Outport  Port=2
  wires:
  v/1 -> hold/1
  hold/1 -> space phasor/1(v)
  t/1 -> space phasor/2(t)
  Vn/1 -> space phasor/3(Vn)
  w0/1 -> space phasor/4(w0)
  space phasor/1(V_re) -> filter/1(re in)
  space phasor/2(V_im) -> filter/2(im in)
  filter/1(re) -> V_re/1
  filter/2(im) -> V_im/1

== system HPP/Network/Network model/Simscape/POC voltage/phasor ==
  v : Inport
  t : Inport  Port=2
  Vn : Constant  Value=p.grid.Vpoc
  filter : Subsystem  Description=Voltage phasor filter, chosen per run by HPP_simscape: None (1, phasor mode) or MAF (2, EMT: moving average over one cycle at p.sim.Ts, starting from the nominal phasor 1 + 0j pu).  Variant=on
  hold : ZeroOrderHold  SampleTime=HPP_Ts
  space phasor : MATLAB Function  TreatAsAtomicUnit=on
  w0 : Constant  Value=2*pi*p.grid.f0
  V_re : Outport
  V_im : Outport  Port=2
  wires:
  v/1 -> hold/1
  hold/1 -> space phasor/1(v)
  t/1 -> space phasor/2(t)
  Vn/1 -> space phasor/3(Vn)
  w0/1 -> space phasor/4(w0)
  space phasor/1(V_re) -> filter/1(re in)
  space phasor/2(V_im) -> filter/2(im in)
  filter/1(re) -> V_re/1
  filter/2(im) -> V_im/1

== system HPP/Network/Network model/Simscape/converter 1/phasor ==
  v : Inport
  t : Inport  Port=2
  Vn : Constant  Value=p.net.wt.Vcol
  filter : Subsystem  Description=Voltage phasor filter, chosen per run by HPP_simscape: None (1, phasor mode) or MAF (2, EMT: moving average over one cycle at p.sim.Ts, starting from the nominal phasor 1 + 0j pu).  Variant=on
  hold : ZeroOrderHold  SampleTime=HPP_Ts
  space phasor : MATLAB Function  TreatAsAtomicUnit=on
  w0 : Constant  Value=2*pi*p.grid.f0
  V_re : Outport
  V_im : Outport  Port=2
  wires:
  v/1 -> hold/1
  hold/1 -> space phasor/1(v)
  t/1 -> space phasor/2(t)
  Vn/1 -> space phasor/3(Vn)
  w0/1 -> space phasor/4(w0)
  space phasor/1(V_re) -> filter/1(re in)
  space phasor/2(V_im) -> filter/2(im in)
  filter/1(re) -> V_re/1
  filter/2(im) -> V_im/1

== system HPP/Network/Network model/Simscape/converter 2/phasor ==
  v : Inport
  t : Inport  Port=2
  Vn : Constant  Value=p.net.wt.Vcol
  filter : Subsystem  Description=Voltage phasor filter, chosen per run by HPP_simscape: None (1, phasor mode) or MAF (2, EMT: moving average over one cycle at p.sim.Ts, starting from the nominal phasor 1 + 0j pu).  Variant=on
  hold : ZeroOrderHold  SampleTime=HPP_Ts
  space phasor : MATLAB Function  TreatAsAtomicUnit=on
  w0 : Constant  Value=2*pi*p.grid.f0
  V_re : Outport
  V_im : Outport  Port=2
  wires:
  v/1 -> hold/1
  hold/1 -> space phasor/1(v)
  t/1 -> space phasor/2(t)
  Vn/1 -> space phasor/3(Vn)
  w0/1 -> space phasor/4(w0)
  space phasor/1(V_re) -> filter/1(re in)
  space phasor/2(V_im) -> filter/2(im in)
  filter/1(re) -> V_re/1
  filter/2(im) -> V_im/1

== system HPP/Network/Network model/Simscape/converter 3/phasor ==
  v : Inport
  t : Inport  Port=2
  Vn : Constant  Value=p.net.pv.Vcol
  filter : Subsystem  Description=Voltage phasor filter, chosen per run by HPP_simscape: None (1, phasor mode) or MAF (2, EMT: moving average over one cycle at p.sim.Ts, starting from the nominal phasor 1 + 0j pu).  Variant=on
  hold : ZeroOrderHold  SampleTime=HPP_Ts
  space phasor : MATLAB Function  TreatAsAtomicUnit=on
  w0 : Constant  Value=2*pi*p.grid.f0
  V_re : Outport
  V_im : Outport  Port=2
  wires:
  v/1 -> hold/1
  hold/1 -> space phasor/1(v)
  t/1 -> space phasor/2(t)
  Vn/1 -> space phasor/3(Vn)
  w0/1 -> space phasor/4(w0)
  space phasor/1(V_re) -> filter/1(re in)
  space phasor/2(V_im) -> filter/2(im in)
  filter/1(re) -> V_re/1
  filter/2(im) -> V_im/1

== system HPP/Network/Network model/Simscape/converter 4/phasor ==
  v : Inport
  t : Inport  Port=2
  Vn : Constant  Value=p.net.pv.Vcol
  filter : Subsystem  Description=Voltage phasor filter, chosen per run by HPP_simscape: None (1, phasor mode) or MAF (2, EMT: moving average over one cycle at p.sim.Ts, starting from the nominal phasor 1 + 0j pu).  Variant=on
  hold : ZeroOrderHold  SampleTime=HPP_Ts
  space phasor : MATLAB Function  TreatAsAtomicUnit=on
  w0 : Constant  Value=2*pi*p.grid.f0
  V_re : Outport
  V_im : Outport  Port=2
  wires:
  v/1 -> hold/1
  hold/1 -> space phasor/1(v)
  t/1 -> space phasor/2(t)
  Vn/1 -> space phasor/3(Vn)
  w0/1 -> space phasor/4(w0)
  space phasor/1(V_re) -> filter/1(re in)
  space phasor/2(V_im) -> filter/2(im in)
  filter/1(re) -> V_re/1
  filter/2(im) -> V_im/1

== system HPP/Network/Network model/Simscape/converter 5/phasor ==
  v : Inport
  t : Inport  Port=2
  Vn : Constant  Value=p.net.bess.Vcol
  filter : Subsystem  Description=Voltage phasor filter, chosen per run by HPP_simscape: None (1, phasor mode) or MAF (2, EMT: moving average over one cycle at p.sim.Ts, starting from the nominal phasor 1 + 0j pu).  Variant=on
  hold : ZeroOrderHold  SampleTime=HPP_Ts
  space phasor : MATLAB Function  TreatAsAtomicUnit=on
  w0 : Constant  Value=2*pi*p.grid.f0
  V_re : Outport
  V_im : Outport  Port=2
  wires:
  v/1 -> hold/1
  hold/1 -> space phasor/1(v)
  t/1 -> space phasor/2(t)
  Vn/1 -> space phasor/3(Vn)
  w0/1 -> space phasor/4(w0)
  space phasor/1(V_re) -> filter/1(re in)
  space phasor/2(V_im) -> filter/2(im in)
  filter/1(re) -> V_re/1
  filter/2(im) -> V_im/1

== system HPP/Network/Network model/Simscape/solver/EMT ==
  solver : nesl_utility/Solver Configuration  PhysicalDomain=network_engine_domain  SubClassName=solver  LeftPortType=input  RightPortType=generic  Tones=[]  Harmonics=[]  SimulateNoise=off  Profile=off  UseLocalSampling=off  EnableSwitchedLinearOptims=on  FrequencyDomain=off  UseCCode=off  RelTol=0.001  AbsTol=0.001  MinStep=1e-09  ToWorkspace=off  RevertToSquareIcSolve=off  NumHomotopyIterations=100  PhasorMode=off  PhasorModeNumHarmonics=1  ConsistencySolver=NEWTON_XTOL_AFTER_FTOL  CanonicalOrdering=CANONICAL  OptimizeIntermediates=OPTIMIZED  IndexReductionMethod=DerivativeReplacement  DoDC=off  ResidualTolerance=1e-09  ConsistencyTolSource=GLOBAL  ConsistencyAbsTol=0.001  ConsistencyRelTol=0.001  ConsistencyTolFactor=0.001  UseLocalSolver=on  LocalSolverChoice=NE_BACKWARD_EULER_ADVANCER  ResolveIndetEquations=on  FunctionEvalNumThread=1  LocalSolverSampleTime=HPP_Tnet  DoFixedCost=on  MaxNonlinIter=1  MaxModeIter=2  ComputeImpulses=off  ImpulseIterations=2  LinearAlgebra=auto  LinearAlgebraNumThread=0  EquationFormulation=NE_TIME_EF  DelaysMemoryBudget=1024  AutomaticFiltering=on  FilteringTimeConstant=0.001  PartitionStorageMethod=AS_NEEDED  PartitionMemoryBudget=1024  PartitionMethod=ROBUST  MultibodyUseLocalSolver=off  MultibodyLocalSolverChoice=ODE1  MultibodyLocalSolverSampleTime=0.001
  ~ : PMIOPort  Side=Right
  connections:
  solver/RConn1 -- ~/RConn1

== system HPP/Network/Network model/Simscape/solver/Phasor ==
  solver : nesl_utility/Solver Configuration  PhysicalDomain=network_engine_domain  SubClassName=solver  LeftPortType=input  RightPortType=generic  Tones=[]  Harmonics=[]  SimulateNoise=off  Profile=off  UseLocalSampling=off  EnableSwitchedLinearOptims=on  FrequencyDomain=off  UseCCode=off  RelTol=0.001  AbsTol=0.001  MinStep=1e-09  ToWorkspace=off  RevertToSquareIcSolve=off  NumHomotopyIterations=100  PhasorMode=off  PhasorModeNumHarmonics=1  ConsistencySolver=NEWTON_XTOL_AFTER_FTOL  CanonicalOrdering=CANONICAL  OptimizeIntermediates=OPTIMIZED  IndexReductionMethod=DerivativeReplacement  DoDC=off  ResidualTolerance=1e-09  ConsistencyTolSource=GLOBAL  ConsistencyAbsTol=0.001  ConsistencyRelTol=0.001  ConsistencyTolFactor=0.001  UseLocalSolver=on  LocalSolverChoice=NE_BACKWARD_EULER_ADVANCER  ResolveIndetEquations=on  FunctionEvalNumThread=1  LocalSolverSampleTime=HPP_Tnet  DoFixedCost=on  MaxNonlinIter=1  MaxModeIter=2  ComputeImpulses=off  ImpulseIterations=2  LinearAlgebra=auto  LinearAlgebraNumThread=0  EquationFormulation=NE_FREQUENCY_TIME_EF  DelaysMemoryBudget=1024  AutomaticFiltering=on  FilteringTimeConstant=0.001  PartitionStorageMethod=AS_NEEDED  PartitionMemoryBudget=1024  PartitionMethod=ROBUST  MultibodyUseLocalSolver=off  MultibodyLocalSolverChoice=ODE1  MultibodyLocalSolverSampleTime=0.001
  ~ : PMIOPort  Side=Right
  connections:
  solver/RConn1 -- ~/RConn1

== system HPP/Network/Network model/Simscape/HPP bus voltage/phasor/filter ==
  note: 1) Add Subsystem or Model blocks as valid variant choices.
      | 2) You cannot connect blocks at this level. At simulation, connectivity is automatically
      | determined, based on the active variant and port name matching.
  re in : Inport
  im in : Inport  Port=2
  MAF : Subsystem  VariantControl=HPP_simscape == 2
  None : Subsystem  VariantControl=HPP_simscape == 1
  re : Outport
  im : Outport  Port=2

== system HPP/Network/Network model/Simscape/POC voltage/phasor/filter ==
  note: 1) Add Subsystem or Model blocks as valid variant choices.
      | 2) You cannot connect blocks at this level. At simulation, connectivity is automatically
      | determined, based on the active variant and port name matching.
  re in : Inport
  im in : Inport  Port=2
  MAF : Subsystem  VariantControl=HPP_simscape == 2
  None : Subsystem  VariantControl=HPP_simscape == 1
  re : Outport
  im : Outport  Port=2

== system HPP/Network/Network model/Simscape/converter 1/phasor/filter ==
  note: 1) Add Subsystem or Model blocks as valid variant choices.
      | 2) You cannot connect blocks at this level. At simulation, connectivity is automatically
      | determined, based on the active variant and port name matching.
  re in : Inport
  im in : Inport  Port=2
  MAF : Subsystem  VariantControl=HPP_simscape == 2
  None : Subsystem  VariantControl=HPP_simscape == 1
  re : Outport
  im : Outport  Port=2

== system HPP/Network/Network model/Simscape/converter 2/phasor/filter ==
  note: 1) Add Subsystem or Model blocks as valid variant choices.
      | 2) You cannot connect blocks at this level. At simulation, connectivity is automatically
      | determined, based on the active variant and port name matching.
  re in : Inport
  im in : Inport  Port=2
  MAF : Subsystem  VariantControl=HPP_simscape == 2
  None : Subsystem  VariantControl=HPP_simscape == 1
  re : Outport
  im : Outport  Port=2

== system HPP/Network/Network model/Simscape/converter 3/phasor/filter ==
  note: 1) Add Subsystem or Model blocks as valid variant choices.
      | 2) You cannot connect blocks at this level. At simulation, connectivity is automatically
      | determined, based on the active variant and port name matching.
  re in : Inport
  im in : Inport  Port=2
  MAF : Subsystem  VariantControl=HPP_simscape == 2
  None : Subsystem  VariantControl=HPP_simscape == 1
  re : Outport
  im : Outport  Port=2

== system HPP/Network/Network model/Simscape/converter 4/phasor/filter ==
  note: 1) Add Subsystem or Model blocks as valid variant choices.
      | 2) You cannot connect blocks at this level. At simulation, connectivity is automatically
      | determined, based on the active variant and port name matching.
  re in : Inport
  im in : Inport  Port=2
  MAF : Subsystem  VariantControl=HPP_simscape == 2
  None : Subsystem  VariantControl=HPP_simscape == 1
  re : Outport
  im : Outport  Port=2

== system HPP/Network/Network model/Simscape/converter 5/phasor/filter ==
  note: 1) Add Subsystem or Model blocks as valid variant choices.
      | 2) You cannot connect blocks at this level. At simulation, connectivity is automatically
      | determined, based on the active variant and port name matching.
  re in : Inport
  im in : Inport  Port=2
  MAF : Subsystem  VariantControl=HPP_simscape == 2
  None : Subsystem  VariantControl=HPP_simscape == 1
  re : Outport
  im : Outport  Port=2

== system HPP/Network/Network model/Simscape/HPP bus voltage/phasor/filter/MAF ==
  re in : Inport
  im in : Inport  Port=2
  MAF im : DiscreteFir  Coefficients=ones(1,round(1/(HPP_f0*HPP_Ts)))/round(1/(HPP_f0*HPP_Ts))
  MAF re : DiscreteFir  Coefficients=ones(1,round(1/(HPP_f0*HPP_Ts)))/round(1/(HPP_f0*HPP_Ts))  InitialStates=1
  re : Outport
  im : Outport  Port=2
  wires:
  re in/1 -> MAF re/1
  MAF re/1 -> re/1
  im in/1 -> MAF im/1
  MAF im/1 -> im/1

== system HPP/Network/Network model/Simscape/HPP bus voltage/phasor/filter/None ==
  re in : Inport
  im in : Inport  Port=2
  re : Outport
  im : Outport  Port=2
  wires:
  re in/1 -> re/1
  im in/1 -> im/1

== system HPP/Network/Network model/Simscape/POC voltage/phasor/filter/MAF ==
  re in : Inport
  im in : Inport  Port=2
  MAF im : DiscreteFir  Coefficients=ones(1,round(1/(HPP_f0*HPP_Ts)))/round(1/(HPP_f0*HPP_Ts))
  MAF re : DiscreteFir  Coefficients=ones(1,round(1/(HPP_f0*HPP_Ts)))/round(1/(HPP_f0*HPP_Ts))  InitialStates=1
  re : Outport
  im : Outport  Port=2
  wires:
  re in/1 -> MAF re/1
  MAF re/1 -> re/1
  im in/1 -> MAF im/1
  MAF im/1 -> im/1

== system HPP/Network/Network model/Simscape/POC voltage/phasor/filter/None ==
  re in : Inport
  im in : Inport  Port=2
  re : Outport
  im : Outport  Port=2
  wires:
  re in/1 -> re/1
  im in/1 -> im/1

== system HPP/Network/Network model/Simscape/converter 1/phasor/filter/MAF ==
  re in : Inport
  im in : Inport  Port=2
  MAF im : DiscreteFir  Coefficients=ones(1,round(1/(HPP_f0*HPP_Ts)))/round(1/(HPP_f0*HPP_Ts))
  MAF re : DiscreteFir  Coefficients=ones(1,round(1/(HPP_f0*HPP_Ts)))/round(1/(HPP_f0*HPP_Ts))  InitialStates=1
  re : Outport
  im : Outport  Port=2
  wires:
  re in/1 -> MAF re/1
  MAF re/1 -> re/1
  im in/1 -> MAF im/1
  MAF im/1 -> im/1

== system HPP/Network/Network model/Simscape/converter 1/phasor/filter/None ==
  re in : Inport
  im in : Inport  Port=2
  re : Outport
  im : Outport  Port=2
  wires:
  re in/1 -> re/1
  im in/1 -> im/1

== system HPP/Network/Network model/Simscape/converter 2/phasor/filter/MAF ==
  re in : Inport
  im in : Inport  Port=2
  MAF im : DiscreteFir  Coefficients=ones(1,round(1/(HPP_f0*HPP_Ts)))/round(1/(HPP_f0*HPP_Ts))
  MAF re : DiscreteFir  Coefficients=ones(1,round(1/(HPP_f0*HPP_Ts)))/round(1/(HPP_f0*HPP_Ts))  InitialStates=1
  re : Outport
  im : Outport  Port=2
  wires:
  re in/1 -> MAF re/1
  MAF re/1 -> re/1
  im in/1 -> MAF im/1
  MAF im/1 -> im/1

== system HPP/Network/Network model/Simscape/converter 2/phasor/filter/None ==
  re in : Inport
  im in : Inport  Port=2
  re : Outport
  im : Outport  Port=2
  wires:
  re in/1 -> re/1
  im in/1 -> im/1

== system HPP/Network/Network model/Simscape/converter 3/phasor/filter/MAF ==
  re in : Inport
  im in : Inport  Port=2
  MAF im : DiscreteFir  Coefficients=ones(1,round(1/(HPP_f0*HPP_Ts)))/round(1/(HPP_f0*HPP_Ts))
  MAF re : DiscreteFir  Coefficients=ones(1,round(1/(HPP_f0*HPP_Ts)))/round(1/(HPP_f0*HPP_Ts))  InitialStates=1
  re : Outport
  im : Outport  Port=2
  wires:
  re in/1 -> MAF re/1
  MAF re/1 -> re/1
  im in/1 -> MAF im/1
  MAF im/1 -> im/1

== system HPP/Network/Network model/Simscape/converter 3/phasor/filter/None ==
  re in : Inport
  im in : Inport  Port=2
  re : Outport
  im : Outport  Port=2
  wires:
  re in/1 -> re/1
  im in/1 -> im/1

== system HPP/Network/Network model/Simscape/converter 4/phasor/filter/MAF ==
  re in : Inport
  im in : Inport  Port=2
  MAF im : DiscreteFir  Coefficients=ones(1,round(1/(HPP_f0*HPP_Ts)))/round(1/(HPP_f0*HPP_Ts))
  MAF re : DiscreteFir  Coefficients=ones(1,round(1/(HPP_f0*HPP_Ts)))/round(1/(HPP_f0*HPP_Ts))  InitialStates=1
  re : Outport
  im : Outport  Port=2
  wires:
  re in/1 -> MAF re/1
  MAF re/1 -> re/1
  im in/1 -> MAF im/1
  MAF im/1 -> im/1

== system HPP/Network/Network model/Simscape/converter 4/phasor/filter/None ==
  re in : Inport
  im in : Inport  Port=2
  re : Outport
  im : Outport  Port=2
  wires:
  re in/1 -> re/1
  im in/1 -> im/1

== system HPP/Network/Network model/Simscape/converter 5/phasor/filter/MAF ==
  re in : Inport
  im in : Inport  Port=2
  MAF im : DiscreteFir  Coefficients=ones(1,round(1/(HPP_f0*HPP_Ts)))/round(1/(HPP_f0*HPP_Ts))
  MAF re : DiscreteFir  Coefficients=ones(1,round(1/(HPP_f0*HPP_Ts)))/round(1/(HPP_f0*HPP_Ts))  InitialStates=1
  re : Outport
  im : Outport  Port=2
  wires:
  re in/1 -> MAF re/1
  MAF re/1 -> re/1
  im in/1 -> MAF im/1
  MAF im/1 -> im/1

== system HPP/Network/Network model/Simscape/converter 5/phasor/filter/None ==
  re in : Inport
  im in : Inport  Port=2
  re : Outport
  im : Outport  Port=2
  wires:
  re in/1 -> re/1
  im in/1 -> im/1

== matlab function HPP/Network/Network model/Simscape/converter 3/phasor/space phasor ==
  data: v input; V_re output; t input; Vn input; w0 input; V_im output
function [V_re, V_im] = phasor(v, t, Vn, w0)
%#codegen
% space phasor at the nominal frequency: exact phasor in frequency-and-time mode;
% in time (EMT) mode the instantaneous space phasor (filtered after this block)
a = complex(-0.5, sqrt(3)/2);
s = 2/3*(v(1) + a*v(2) + a^2*v(3)) * exp(complex(0, pi/2 - w0*t));
V = s * sqrt(3/2) / Vn;
V_re = real(V);
V_im = imag(V);
end
